simulink library "Model_DG_Synchronous_Generator"  (R2022b)
settings: Solver=VariableStepAuto  StartTime=0.0  StopTime=10.0  RelTol=1e-3
libraries: eeGeneralControl x11, simulink x6, slpidlib x4, spsPositiveSequencePLLDrivenLib x3, spsAC1AExcitationSystemLib x1, spsAC4AExcitationSystemLib x1, spsAC5AExcitationSystemLib x1, spsDC1AExcitationSystemLib x1, spsDC2AExcitationSystemLib x1, spsST1AExcitationSystemLib x1, spsST2AExcitationSystemLib x1, spsPLL3phLib x1
(part 2 of 2)

== system Model_DG_Synchronous_Generator/Synchronous_Generator/SG_Control/Reactive_Power_Controller/Constant_Voltage ==
  mode : Inport
  V_grid_pu : Inport  Port=2
  Q_set_pu : Inport  Port=3
  P_grid_pu : Inport  Port=4
  Q_grid_pu : Inport  Port=5
  Constant : Constant  Value=0
  Terminator{,1..4} (5 alike) : Terminator
  V_stab_pu : Outport
  wires:
  mode/1 -> Terminator/1
  V_grid_pu/1 -> Terminator1/1
  Q_set_pu/1 -> Terminator2/1
  P_grid_pu/1 -> Terminator3/1
  Q_grid_pu/1 -> Terminator4/1
  Constant/1 -> V_stab_pu/1

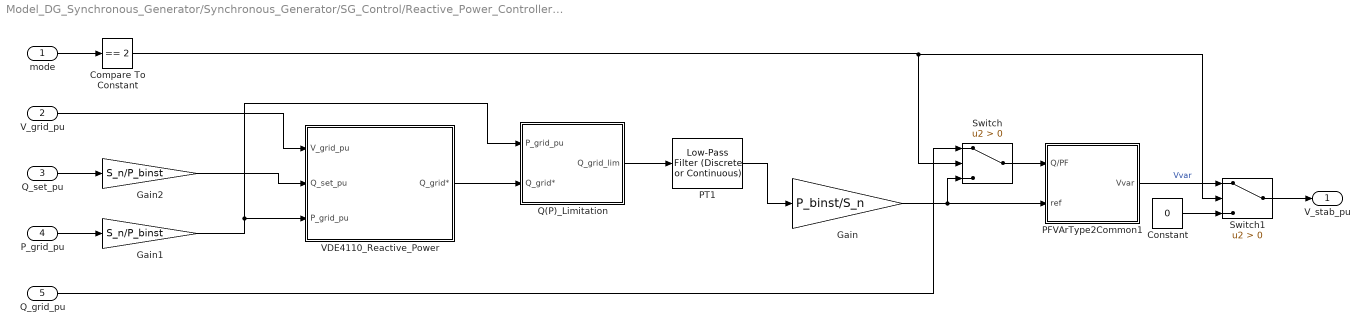
== system Model_DG_Synchronous_Generator/Synchronous_Generator/SG_Control/Reactive_Power_Controller/Reactive_Power_Control ==
  mode : Inport
  V_grid_pu : Inport  Port=2
  Q_set_pu : Inport  Port=3
  P_grid_pu : Inport  Port=4
  Q_grid_pu : Inport  Port=5
  Compare To Constant : simulink/Logic and Bit Operations/Compare To Constant  relop===  const=2  OutDataTypeStr=boolean
  Constant : Constant  Value=0
  Gain : Gain  Gain=P_binst/S_n
  Gain1 : Gain  Gain=S_n/P_binst
  Gain2 : Gain  Gain=S_n/P_binst
  PFVArType2Common1 : Subsystem  mask(PFVArType2Common1){kp=K_p_QCtrl, ki=K_i_QCtrl, max=1}
      mask prompts: kp "Proportionalverstärkung (Kp)"; ki "Rückstellverstärkung (Ki)"; max "Begrenzung des Ausgangs (max)"
      mask help:
      | Leistungsfaktor-/Blindleistungsregler. Diese Modell stellt einen Leistungsfaktor- oder Blindleistungsregler wie
      | den Basler SCP-250 dar. Der Regler misst Leistungsfaktor oder Blindleistung (PU der Bemessungsleistung
      | des Generators) und vergleicht diesen bzw. diese mit dem Sollwert des Bedieners.
      | [Fußnote: Basler SCP-250 ist ein Beispiel für ein handelsübliches Produkt. Diese Angabe dient nur zur
      | Unterrichtung der Anwender dieses Dokuments und bedeutet keine Anerkennung dieses genannten Produkts
      | durch IEC.]
  PT1 : eeGeneralControl/Low-Pass Filter (Discrete or Continuous)  K=1  T=10/3  B=inf  A=-inf  init_option=Inherited from block input  x0=0  Ts=-1
  Q(P)_Limitation : Subsystem
  Switch : Switch  Criteria=u2 > Threshold  SaturateOnIntegerOverflow=off  InputSameDT=off
  Switch1 : Switch  Criteria=u2 > Threshold  SaturateOnIntegerOverflow=off  InputSameDT=off
  VDE4110_Reactive_Power : Subsystem  Variant=on  VariantControl=Choice
  V_stab_pu : Outport
  wires:
  PFVArType2Common1/1(Vvar) -> Switch1/1  "Vvar"
  Q_set_pu/1 -> Gain2/1
  Q_grid_pu/1 -> Switch/1
  Q(P)_Limitation/1(Q_grid_lim) -> PT1/1
  Gain/1 -> PFVArType2Common1/2(ref), Switch/3
  V_grid_pu/1 -> VDE4110_Reactive_Power/1(V_grid_pu)
  P_grid_pu/1 -> Gain1/1
  Gain2/1 -> VDE4110_Reactive_Power/2(Q_set_pu)
  VDE4110_Reactive_Power/1(Q_grid*) -> Q(P)_Limitation/2(Q_grid*)
  mode/1 -> Compare To Constant/1
  PT1/1 -> Gain/1
  Constant/1 -> Switch1/3
  Gain1/1 -> Q(P)_Limitation/1(P_grid_pu), VDE4110_Reactive_Power/3(P_grid_pu)
  Switch1/1 -> V_stab_pu/1
  Switch/1 -> PFVArType2Common1/1(Q/PF)
  Compare To Constant/1 -> Switch1/2, Switch/2

== system Model_DG_Synchronous_Generator/Synchronous_Generator/SG_Control/Reactive_Power_Controller/Reactive_Power_Control/PFVArType2Common1 ==
  Q/PF : Inport
  ref : Inport  Port=2
  PID Controller : slpidlib/PID Controller  Controller=PI  Form=Parallel  TimeDomain=Discrete-time  UseExternalTs=off  SampleTime=-1  IntegratorMethod=Forward Euler  FilterMethod=Forward Euler  ControllerParametersSource=internal  P=kp  I=ki  D=0  UseFilter=on  N=100  TunerSelectOption=Transfer Function Based (PID Tuner App)  InitialConditionSource=internal  InitialConditionForIntegrator=0  InitialConditionForFilter=0  DifferentiatorICPrevScaledInput=0  ExternalReset=none  TrackingMode=off  Kt=1  LimitOutput=on  SatLimitsSource=internal  UpperSaturationLimit=max  LowerSaturationLimit=-max  LinearizeAsGain=on  AntiWindupMode=none  Kb=1  POutMin=[]  POutMax=[]  IOutMin=[]  IOutMax=[]  DOutMin=[]  DOutMax=[]  NOutMin=[]  NOutMax=[]  SumOutMin=[]  SumOutMax=[]  SaturationOutMin=[]  SaturationOutMax=[]  PParamMin=[]  PParamMax=[]  IParamMin=[]  IParamMax=[]  DParamMin=[]  DParamMax=[]  NParamMin=[]  NParamMax=[]  KbParamMin=[]  KbParamMax=[]  KtParamMin=[]  KtParamMax=[]  KbOutMin=[]  KbOutMax=[]  KtOutMin=[]  KtOutMax=[]  IntegratorOutMin=[]  IntegratorOutMax=[]  FilterOutMin=[]  FilterOutMax=[]  SumI1OutMin=[]  SumI1OutMax=[]  SumI2OutMin=[]  SumI2OutMax=[]  SumI3OutMin=[]  SumI3OutMax=[]  SumI4OutMin=[]  SumI4OutMax=[]  SumDOutMin=[]  SumDOutMax=[]  DifferentiatorOutMin=[]  DifferentiatorOutMax=[]  FilterDiffOutCoefMin=[]  FilterDiffOutCoefMax=[]  ReciprocalOutMin=[]  ReciprocalOutMax=[]  SumDenOutMin=[]  SumDenOutMax=[]  SumNumOutMin=[]  SumNumOutMax=[]  DivideOutMin=[]  DivideOutMax=[]  UdiffTsProdOutMin=[]  UdiffTsProdOutMax=[]  NTsProdOutMin=[]  NTsProdOutMax=[]  UintegralTsProdOutMin=[]  UintegralTsProdOutMax=[]  UngainTsProdOutMin=[]  UngainTsProdOutMax=[]  FilterDenConstantOutDataTypeStr=Inherit: Inherit via back propagation  FilterDenConstantOutMin=[]  FilterDenConstantOutMax=[]  PCopyOutDataTypeStr=Inherit: Inherit via back propagation  PCopyOutMin=[]  PCopyOutMax=[]  NCopyOutDataTypeStr=Inherit: Inherit via back propagation  NCopyOutMin=[]  NCopyOutMax=[]  IntegratorContinuousStateAttributes=''  IntegratorStateMustResolveToSignalObject=off  IntegratorRTWStateStorageClass=Auto  FilterContinuousStateAttributes=''  FilterStateMustResolveToSignalObject=off  FilterRTWStateStorageClass=Auto  ParallelPVariant=InternalParameters  IdealPVariant=Disabled  IVariant=InternalParameters  DVariant=Disabled  IntegratorVariant=Discrete  SatVariant=Enabled  AWVariant=Passthrough  PCopyVariant=Disabled  TRVariant=Disabled  FdbkBlocksVariant=Forward  IdealPFdbkVariant=Disabled  SatFdbkVariant=Disabled  DerivativeFilterVariant=Disabled  NVariant=Disabled  NCopyVariant=Disabled_SignalSpec  FilterICVariant=Disabled  IntegratorICVariant=InternalICs  ExternalResetVariant=Disabled  TRSumVariant=Passthrough  SumFdbkVariant=Disabled  SumVariant=Sum_PI  TsampFilterVariant=InternalTs  TsampNgainVariant=Passthrough  TsampIntegralVariant=Passthrough  ExternalSaturationOutDataTypeStr=Inherit: Same as second input
  Sum : Sum  Inputs=|-+
  Vvar : Outport  VectorParamsAs1DForOutWhenUnconnected=off
  wires:
  Q/PF/1 -> Sum/1
  PID Controller/1 -> Vvar/1
  ref/1 -> Sum/2
  Sum/1 -> PID Controller/1

== system Model_DG_Synchronous_Generator/Synchronous_Generator/SG_Control/Reactive_Power_Controller/Reactive_Power_Control/Q(P)_Limitation ==
  P_grid_pu : Inport
  Q_grid* : Inport  Port=2
  Add : Sum
  Add1 : Sum  Inputs=-+|
  Compare To Constant : simulink/Logic and Bit Operations/Compare To Constant  relop=>=  const=0.2  OutDataTypeStr=uint8
  Compare To Constant1 : simulink/Logic and Bit Operations/Compare To Constant  relop=>=  const=0.1  OutDataTypeStr=uint8
  Constant : Constant  Value=0.13
  Gain : Gain  Gain=2.3
  Gain1 : Gain  Gain=-1
  Multiport Switch : MultiPortSwitch  DataPortOrder=Zero-based contiguous  zeroidx=on  SaturateOnIntegerOverflow=off  InputSameDT=off
  Saturation : Saturate  UpperLimit=0.33  LowerLimit=-0.33
  Saturation Dynamic : simulink/Discontinuities/Saturation Dynamic  OutMin=[]  OutMax=[]  OutDataTypeStr=Inherit: Same as second input  OutDataType=fixdt(1, 16)  OutScaling=2^-10  DoSatur=off
  Saturation1 : Saturate  UpperLimit=0.02  LowerLimit=-0.05
  Q_grid_lim : Outport
  wires:
  Compare To Constant/1 -> Add/1
  Compare To Constant1/1 -> Add/2
  Add/1 -> Multiport Switch/1
  Saturation/1 -> Multiport Switch/4
  Saturation1/1 -> Multiport Switch/2
  Q_grid*/1 -> Saturation Dynamic/2, Saturation/1, Saturation1/1
  Multiport Switch/1 -> Q_grid_lim/1
  Saturation Dynamic/1 -> Multiport Switch/3
  Gain/1 -> Add1/2
  Constant/1 -> Add1/1
  Add1/1 -> Saturation Dynamic/1, Gain1/1
  Gain1/1 -> Saturation Dynamic/3
  P_grid_pu/1 -> Gain/1, Compare To Constant1/1, Compare To Constant/1

== system Model_DG_Synchronous_Generator/Synchronous_Generator/SG_Control/Reactive_Power_Controller/Reactive_Power_Control/VDE4110_Reactive_Power ==
  V_grid_pu : Inport
  Q_set_pu : Inport  Port=2
  P_grid_pu : Inport  Port=3
  (a)_Q(V) : Subsystem  VariantControl=QCtrl == 2
  (b)_Q(P) : Subsystem  VariantControl=QCtrl == 3
  (c)_Q(V)_with_const_Q : Subsystem  VariantControl=QCtrl == 4
  (d)_cos_phi : Subsystem  VariantControl=(default)
  Q_grid* : Outport

== system Model_DG_Synchronous_Generator/Synchronous_Generator/SG_Control/Reactive_Power_Controller/Reactive_Power_Control/VDE4110_Reactive_Power/(a)_Q(V) ==
  V_grid_pu : Inport
  Q_set_pu : Inport  Port=2
  P_grid_pu : Inport  Port=3
  Q(V)_curve : Subsystem  mask{deadband=deadband, umax=umax, qmax=qmax, uq0ref=uq0ref}
      mask prompts: deadband "Voltage Deadband [+- %]"; umax "U_max [pu]"; qmax "|Q_max| [pu]"; uq0ref "U_Q0ref [pu]"
      mask DialogControl DescGroupVar Prompt: Q(V)-curve
      mask DialogControl DescTextVar Prompt: Q(V)-curve according to VDE 4110. Detailed parameter descriptions are given in the VDE 4110 document.
  Terminator : Terminator
  Terminator1 : Terminator
  Q_grid* : Outport
  wires:
  V_grid_pu/1 -> Q(V)_curve/1(V_grid)
  Q(V)_curve/1(Q_grid*) -> Q_grid*/1
  Q_set_pu/1 -> Terminator/1
  P_grid_pu/1 -> Terminator1/1

== system Model_DG_Synchronous_Generator/Synchronous_Generator/SG_Control/Reactive_Power_Controller/Reactive_Power_Control/VDE4110_Reactive_Power/(b)_Q(P) ==
  V_grid_pu : Inport
  Q_set_pu : Inport  Port=2
  P_grid_pu : Inport  Port=3
  Q(P)-curve : Subsystem  mask{q_pu=q_pu, p_pu=p_pu}
      mask prompts: q_pu "Q_grid points [pu]"; p_pu "P_grid points [pu]"
      mask DialogControl DescGroupVar Prompt: Q(P)-curve
      mask DialogControl DescTextVar Prompt: Q(P)-curve according to VDE 4110. Detailed parameter descriptions are given in the VDE 4110 document.
      mask DialogControl Control2 Prompt: In contrast to VDE 4110, here the active and reactive power values are given in active sign convention.
  Terminator : Terminator
  Terminator1 : Terminator
  Q_grid* : Outport
  wires:
  P_grid_pu/1 -> Q(P)-curve/1(P_grid)
  V_grid_pu/1 -> Terminator/1
  Q_set_pu/1 -> Terminator1/1
  Q(P)-curve/1(Q_grid*) -> Q_grid*/1

== system Model_DG_Synchronous_Generator/Synchronous_Generator/SG_Control/Reactive_Power_Controller/Reactive_Power_Control/VDE4110_Reactive_Power/(c)_Q(V)_with_const_Q ==
  V_grid_pu : Inport
  Q_set_pu : Inport  Port=2
  P_grid_pu : Inport  Port=3
  Q(V)_with_const_Q : Subsystem  mask{p1=p1, p2=p2, p3=p3, p4=p4}
      mask prompts: p1 "P1 [V_grid, Q_grid] [pu]"; p2 "P2 [V_grid, Q_grid] [pu]"; p3 "P3 [V_grid, Q_grid] [pu]"; p4 "P4 [V_grid, Q_grid] [pu]"
      mask DialogControl DescGroupVar Prompt: Constant Q with voltage limitation
      mask DialogControl DescTextVar Prompt: Q(V)-curve according to VDE 4110. Detailed parameter descriptions are given in the VDE 4110 document.
      mask DialogControl Control2 Prompt: In contrast to VDE 4110, here the reactive power values are given in active sign convention.
  Terminator : Terminator
  Q_grid* : Outport
  wires:
  V_grid_pu/1 -> Q(V)_with_const_Q/1(V_grid)
  Q_set_pu/1 -> Q(V)_with_const_Q/2(Q_set)
  P_grid_pu/1 -> Terminator/1
  Q(V)_with_const_Q/1(Q_grid*) -> Q_grid*/1

== system Model_DG_Synchronous_Generator/Synchronous_Generator/SG_Control/Reactive_Power_Controller/Reactive_Power_Control/VDE4110_Reactive_Power/(d)_cos_phi ==
  V_grid_pu : Inport
  Q_set_pu : Inport  Port=2
  P_grid_pu : Inport  Port=3
  Constant_cos_phi : Subsystem  mask{cosphi_ref=cosphi_ref, ind_cap_Q=ind_cap_Q}
      mask prompts: cosphi_ref "cos(phi)"
      mask DialogControl DescGroupVar Prompt: Constant cos(phi)
      mask DialogControl DescTextVar Prompt: Constant cos(phi) behavior according to VDE 4110. Detailed parameter descriptions are given in the VDE 4110 document.
  Terminator : Terminator
  Terminator1 : Terminator
  Q_grid* : Outport
  wires:
  Constant_cos_phi/1(Q_grid*) -> Q_grid*/1
  P_grid_pu/1 -> Constant_cos_phi/1(P_grid)
  V_grid_pu/1 -> Terminator/1
  Q_set_pu/1 -> Terminator1/1

== system Model_DG_Synchronous_Generator/Synchronous_Generator/SG_Control/Reactive_Power_Controller/Reactive_Power_Control/VDE4110_Reactive_Power/(a)_Q(V)/Q(V)_curve ==
  V_grid : Inport
  Constant : Constant  Value=uq0ref
  Dead Zone : DeadZone  LowerValue=-deadband/100  UpperValue=+deadband/100
  Gain : Gain  Gain=qmax/(umax-uq0ref)
  Saturation : Saturate  UpperLimit=qmax  LowerLimit=-qmax
  Sum : Sum  Inputs=|-+
  Q_grid* : Outport  VectorParamsAs1DForOutWhenUnconnected=off
  wires:
  Constant/1 -> Sum/2
  Saturation/1 -> Q_grid*/1
  Dead Zone/1 -> Gain/1
  Gain/1 -> Saturation/1
  Sum/1 -> Dead Zone/1
  V_grid/1 -> Sum/1

== system Model_DG_Synchronous_Generator/Synchronous_Generator/SG_Control/Reactive_Power_Controller/Reactive_Power_Control/VDE4110_Reactive_Power/(b)_Q(P)/Q(P)-curve ==
  P_grid : Inport
  1-D Lookup Table : Lookup_n-D  NumberOfTableDimensions=1  BreakpointsForDimension1=p_pu  Table=q_pu  InternalRulePriority=Speed  RndMeth=Simplest
  Q_grid* : Outport  VectorParamsAs1DForOutWhenUnconnected=off
  wires:
  1-D Lookup Table/1 -> Q_grid*/1
  P_grid/1 -> 1-D Lookup Table/1

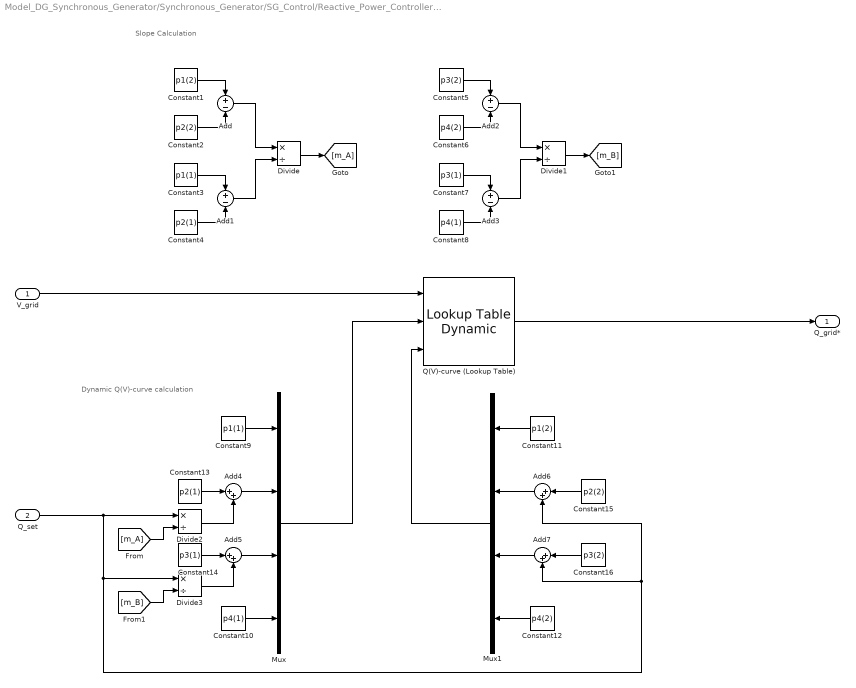
== system Model_DG_Synchronous_Generator/Synchronous_Generator/SG_Control/Reactive_Power_Controller/Reactive_Power_Control/VDE4110_Reactive_Power/(c)_Q(V)_with_const_Q/Q(V)_with_const_Q ==
  note: Dynamic Q(V)-curve calculation
  note: Slope Calculation
  V_grid : Inport
  Q_set : Inport  Port=2
  Add{,1..3} (4 alike) : Sum  Inputs=+|-
  Add{4..7} (4 alike) : Sum  Inputs=|++
  Constant1 : Constant  Value=p1(2)
  Constant10 : Constant  Value=p4(1)
  Constant11 : Constant  Value=p1(2)
  Constant12 : Constant  Value=p4(2)
  Constant13 : Constant  Value=p2(1)
  Constant14 : Constant  Value=p3(1)
  Constant15 : Constant  Value=p2(2)
  Constant16 : Constant  Value=p3(2)
  Constant2 : Constant  Value=p2(2)
  Constant3 : Constant  Value=p1(1)
  Constant4 : Constant  Value=p2(1)
  Constant5 : Constant  Value=p3(2)
  Constant6 : Constant  Value=p4(2)
  Constant7 : Constant  Value=p3(1)
  Constant8 : Constant  Value=p4(1)
  Constant9 : Constant  Value=p1(1)
  Divide{,1..3} (4 alike) : Product  Inputs=*/
  Mux : Mux
  Mux1 : Mux
  Q(V)-curve (Lookup Table) : simulink/Lookup Tables/Lookup Table Dynamic  LookUpMeth=Interpolation-Use End Values  OutDataType=fixdt('double')  OutScaling=[]  OutputDataTypeScalingMode=Specify via dialog  OutDataTypeStr=double  DoSatur=off
  Q_grid* : Outport  VectorParamsAs1DForOutWhenUnconnected=off
  wires:
  V_grid/1 -> Q(V)-curve (Lookup Table)/1
  Q(V)-curve (Lookup Table)/1 -> Q_grid*/1
  Constant1/1 -> Add/1
  Constant2/1 -> Add/2
  Constant4/1 -> Add1/2
  Constant3/1 -> Add1/1
  Add/1 -> Divide/1
  Add1/1 -> Divide/2
  Divide/1 -> [m_A]
  Divide1/1 -> [m_B]
  Constant7/1 -> Add3/1
  Add2/1 -> Divide1/1
  Constant8/1 -> Add3/2
  Add3/1 -> Divide1/2
  Constant6/1 -> Add2/2
  Constant5/1 -> Add2/1
  Constant9/1 -> Mux/1
  Constant10/1 -> Mux/4
  Mux/1 -> Q(V)-curve (Lookup Table)/2
  Mux1/1 -> Q(V)-curve (Lookup Table)/3
  Constant11/1 -> Mux1/1
  Constant12/1 -> Mux1/4
  Add5/1 -> Mux/3
  Add4/1 -> Mux/2
  Constant13/1 -> Add4/1
  Constant14/1 -> Add5/1
  Divide2/1 -> Add4/2
  Divide3/1 -> Add5/2
  [m_A] -> Divide2/2
  [m_B] -> Divide3/2
  Add6/1 -> Mux1/2
  Add7/1 -> Mux1/3
  Constant16/1 -> Add7/1
  Constant15/1 -> Add6/1
  Q_set/1 -> Add7/2, Add6/2, Divide3/1, Divide2/1

== system Model_DG_Synchronous_Generator/Synchronous_Generator/SG_Control/Reactive_Power_Controller/Reactive_Power_Control/VDE4110_Reactive_Power/(d)_cos_phi/Constant_cos_phi ==
  P_grid : Inport
  Constant : Constant  Value=ind_cap_Q
  Gain : Gain  Gain=tan(acos(cosphi_ref))
  Gain1 : Gain  Gain=-1
  Switch : Switch  Criteria=u2 > Threshold  Threshold=1.5  SaturateOnIntegerOverflow=off  InputSameDT=off
  Q_grid* : Outport  VectorParamsAs1DForOutWhenUnconnected=off
  wires:
  Gain/1 -> Gain1/1, Switch/1
  P_grid/1 -> Gain/1
  Constant/1 -> Switch/2
  Gain1/1 -> Switch/3
  Switch/1 -> Q_grid*/1
